simulink model "LunarMicrogrid_Full"  (R2026b)
settings: Solver=ode23t  StopTime=simulation.timeSim  MaxStep=1/(5*solarPlant.converterSwitchingFrequency)  AbsTol=1e-3
PreLoadFcn:
  | run('LunarMicrogridA_Data');
values from neighbouring files (symbols this model uses):
  Csc = Csc_cell/Ns_sc*Np_sc    (= 200)    [LunarDAB_Params.m]
  eta_sc = 0.95    [LunarDAB_Params.m]
  fsw = 100e3    (= 100000)    [LunarDAB_Params.m]
  k_restore = 1    [LunarDAB_Params.m]
  kiCurrent = 2    [LunarDAB_Params.m]
  kiVoltage = 8    [LunarDAB_Params.m]
  kpCurrent = 0.005    [LunarDAB_Params.m]
  kpVoltage = 0.4    [LunarDAB_Params.m]
  lTotal = lSeries + Llk    [LunarDAB_Params.m]
  P170_dt = 1e-4    (= 0.0001)    [P170_PV_Initialize.m]
  P170_Imp = im(ix)    [P170_PV_Initialize.m]
  P170_Vmp = vm(ix)    [P170_PV_Initialize.m]
  Rd_bat = dV_droop/Ibat_max    (= 0.232258064516)    [LunarDAB_Params.m]
  SC_enable = 1    [LunarDAB_Params.m]
  thetaIC = 0    [LunarDAB_Params.m]
  thetaMaxDab = pi/4    (= 0.785398163397)    [LunarDAB_Params.m]
  Tsw = 1/fsw    (= 1e-05)    [LunarDAB_Params.m]
  Vsc0 = sqrt((Vsc_max^2 + Vsc_min^2)/2)    [LunarDAB_Params.m]
  Vsc_max = 119    [LunarDAB_Params.m]
  Vsc_min = 66    [LunarDAB_Params.m]
undefined symbols (not defined in the file or in its folder): a_lpf_sys, battery, bms, connectedLoad, dcVoltage, DiscIntNeverNeededParam, eta_dab, Ibat_sign, mmc, Ndab, P170_T, pvDroop, sc, sensor, socLimit, solarPlant
libraries: sl_discontinuities x13, fl_lib x13, nesl_utility x13, simulink x7, batteryecm_lib x1, simulink_extras x1, ee_lib x1
(part 7 of 8)

== system LunarMicrogrid_Full/BESS Controller/PIctrl/Filter/Disc. Forward Euler Filter ==
  U : Inport  SampleTime=SampleTime
  Nout : Inport  Port=2  SampleTime=SampleTime
  Reset : Inport  Port=3  SampleTime=SampleTime
  D0in : Inport  Port=4  SampleTime=SampleTime
  N : Inport  Port=5  SampleTime=SampleTime
  Ts : Inport  Port=6  SampleTime=SampleTime
  Filter : DiscreteIntegrator  DisableCoverage=on  SampleTime=SampleTime  OutMin=FilterOutMin  OutMax=FilterOutMax  RndMeth=Simplest  ICPrevOutput=DiscIntNeverNeededParam  ICPrevScaledInput=DiscIntNeverNeededParam
  Signal Specification2 : SignalSpecification  DisableCoverage=on  OutDataTypeStr=boolean  SampleTime=SampleTime
  SumD : Sum  DisableCoverage=on  Inputs=|+-  OutMin=SumDOutMin  OutMax=SumDOutMax  RndMeth=Simplest
  Terminator{,1..3} (4 alike) : Terminator
  Y : Outport  SampleTime=SampleTime
  wires:
  Ts/1 -> Terminator3/1
  D0in/1 -> Terminator/1
  SumD/1 -> Y/1
  Nout/1 -> Filter/1
  U/1 -> SumD/1
  Filter/1 -> SumD/2
  N/1 -> Signal Specification2/1
  Signal Specification2/1 -> Terminator2/1
  Reset/1 -> Terminator1/1

== system LunarMicrogrid_Full/BESS Controller/PIctrl/Filter/Disc. Forward Euler Filter Only ==
  U : Inport  SampleTime=SampleTime
  Nout : Inport  Port=2  SampleTime=SampleTime
  Reset : Inport  Port=3  SampleTime=SampleTime
  D0in : Inport  Port=4  SampleTime=SampleTime
  N : Inport  Port=5  SampleTime=SampleTime
  Ts : Inport  Port=6  SampleTime=SampleTime
  Filter : DiscreteIntegrator  DisableCoverage=on  InitialCondition=InitialConditionForFilter  SampleTime=SampleTime  OutMin=FilterOutMin  OutMax=FilterOutMax  ICPrevOutput=DiscIntNeverNeededParam  ICPrevScaledInput=DiscIntNeverNeededParam
  Signal Specification2 : SignalSpecification  DisableCoverage=on  OutDataTypeStr=boolean  SampleTime=SampleTime
  SumD : Sum  DisableCoverage=on  Inputs=|+-  OutMin=SumDOutMin  OutMax=SumDOutMax
  Terminator{,1..3} (4 alike) : Terminator
  Y : Outport  SampleTime=SampleTime
  wires:
  Filter/1 -> Y/1
  Reset/1 -> Terminator1/1
  Signal Specification2/1 -> Terminator2/1
  N/1 -> Signal Specification2/1
  Nout/1 -> SumD/2
  U/1 -> SumD/1
  SumD/1 -> Filter/1
  D0in/1 -> Terminator/1
  Ts/1 -> Terminator3/1

== system LunarMicrogrid_Full/BESS Controller/PIctrl/Filter/Disc. Trapezoidal Filter ==
  note: Denominator Coefficients
  U : Inport  SampleTime=SampleTime
  N : Inport  Port=2  SampleTime=SampleTime
  Reset : Inport  Port=3  SampleTime=SampleTime
  D0in : Inport  Port=4  SampleTime=SampleTime
  Nout : Inport  Port=5  SampleTime=SampleTime
  Ts : Inport  Port=6  SampleTime=SampleTime
  DenCoefOut : Product  OutMin=FilterDiffOutCoefMin  OutMax=FilterDiffOutCoefMax  RndMeth=Simplest  SampleTime=SampleTime
  Divide : Product  InputSameDT=on  OutMin=DivideOutMin  OutMax=DivideOutMax  RndMeth=Simplest  SampleTime=SampleTime
  Filter Den Constant : Constant  DisableCoverage=on  OutMin=FilterDenConstantOutMin  OutMax=FilterDenConstantOutMax  OutDataTypeStr=Inherit: Inherit via back propagation  PreserveConstantTs=on
  Filter Differentiator TF : DiscreteTransferFcn  Numerator=[1 -1]  DenominatorSource=Input port  SampleTime=SampleTime  a0EqualsOne=on  RndMeth=Simplest
      settings: InputPortMap=u0,p3
  Mux : Mux  Inputs=2
  Passthrough for tuning : DataTypeConversion  Tag=#GainSurfaceTarget_  RndMeth=Simplest  SaturateOnIntegerOverflow=off
  Reciprocal : Math  Operator=reciprocal  OutMin=ReciprocalOutMin  OutMax=ReciprocalOutMax  RndMeth=Simplest  SaturateOnIntegerOverflow=off  OutDataTypeStr=Inherit: Inherit via internal rule
  SumDen : Sum  Inputs=++|  OutMin=SumDenOutMin  OutMax=SumDenOutMax  InputSameDT=on  RndMeth=Simplest
  SumNum : Sum  Inputs=-+|  OutMin=SumNumOutMin  OutMax=SumNumOutMax  InputSameDT=on  RndMeth=Simplest
  Terminator : Terminator
  Terminator1 : Terminator
  Terminator2 : Terminator
  Tsamp : Subsystem  Variant=on  VariantControlMode=label  LabelModeActiveChoice=InternalTs
  Y : Outport  SampleTime=SampleTime
  wires:
  Ts/1 -> Tsamp/2(Ts)
  D0in/1 -> Terminator/1
  Passthrough for tuning/1 -> Tsamp/1(N)
  Tsamp/1(Out1) -> SumDen/2, SumNum/2
  Filter Den Constant/1 -> SumNum/1, Mux/1, SumDen/1
  SumDen/1 -> Reciprocal/1
  SumNum/1 -> Divide/2
  Divide/1 -> Mux/2
  Reciprocal/1 -> DenCoefOut/2, Divide/1
  U/1 -> Filter Differentiator TF/1
  Filter Differentiator TF/1 -> DenCoefOut/1
  Mux/1 -> Filter Differentiator TF/2
  N/1 -> Passthrough for tuning/1
  DenCoefOut/1 -> Y/1
  Nout/1 -> Terminator2/1
  Reset/1 -> Terminator1/1

== system LunarMicrogrid_Full/BESS Controller/PIctrl/Filter/Disc. Trapezoidal Filter Only ==
  note: Denominator Coefficients
  U : Inport  SampleTime=SampleTime
  N : Inport  Port=2  SampleTime=SampleTime
  Reset : Inport  Port=3  SampleTime=SampleTime
  D0in : Inport  Port=4  SampleTime=SampleTime
  Nout : Inport  Port=5  SampleTime=SampleTime
  Ts : Inport  Port=6  SampleTime=SampleTime
  DenCoefOut : Product  OutMin=FilterDiffOutCoefMin  OutMax=FilterDiffOutCoefMax  SampleTime=SampleTime
  Filter Den Constant : Constant  DisableCoverage=on  Value=2  OutMin=FilterDenConstantOutMin  OutMax=FilterDenConstantOutMax  OutDataTypeStr=Inherit: Inherit via back propagation  PreserveConstantTs=on
  Filter Differentiator TF : DiscreteTransferFcn  Numerator=[1 1]  DenominatorSource=Input port  InitialStates=InitialConditionForFilter  SampleTime=SampleTime  a0EqualsOne=on
      settings: InputPortMap=u0,p3
  Mux : Mux  Inputs=2
  Passthrough for tuning : DataTypeConversion  Tag=#GainSurfaceTarget_  SaturateOnIntegerOverflow=off  RndMeth=Floor
  SumDen : Sum  Inputs=|++  OutMin=SumDenOutMin  OutMax=SumDenOutMax  InputSameDT=on
  SumNum : Sum  Inputs=-+|  OutMin=SumNumOutMin  OutMax=SumNumOutMax  InputSameDT=on
  Terminator : Terminator
  Terminator1 : Terminator
  Terminator2 : Terminator
  Tsamp : Subsystem  Variant=on  VariantControlMode=label  LabelModeActiveChoice=InternalTs
  Y : Outport  SampleTime=SampleTime
  wires:
  SumNum/1 -> Mux/2
  SumDen/1 -> Mux/1
  Filter Den Constant/1 -> SumDen/1, SumNum/1
  Tsamp/1(Out1) -> SumDen/2, SumNum/2, DenCoefOut/2
  Reset/1 -> Terminator1/1
  Nout/1 -> Terminator2/1
  DenCoefOut/1 -> Y/1
  N/1 -> Passthrough for tuning/1
  Mux/1 -> Filter Differentiator TF/2
  Filter Differentiator TF/1 -> DenCoefOut/1
  U/1 -> Filter Differentiator TF/1
  Passthrough for tuning/1 -> Tsamp/1(N)
  D0in/1 -> Terminator/1
  Ts/1 -> Tsamp/2(Ts)

== system LunarMicrogrid_Full/BESS Controller/PIctrl/Filter/Passthrough ==
  Reset : Inport  SampleTime=SampleTime
  U : Inport  Port=2  SampleTime=SampleTime
  N : Inport  Port=3  SampleTime=SampleTime
  D0in : Inport  Port=4  SampleTime=SampleTime
  Nout : Inport  Port=5  SampleTime=SampleTime
  Ts : Inport  Port=6  SampleTime=SampleTime
  Signal Specification1 : SignalSpecification  DisableCoverage=on  OutDataTypeStr=boolean  SampleTime=SampleTime
  Signal Specification4 : SignalSpecification  DisableCoverage=on  OutDataTypeStr=boolean  SampleTime=SampleTime
  Terminator{1..2,4..6} (5 alike) : Terminator
  Y : Outport  SampleTime=SampleTime
  wires:
  Nout/1 -> Terminator2/1
  Reset/1 -> Terminator5/1
  D0in/1 -> Signal Specification4/1
  Signal Specification4/1 -> Terminator4/1
  N/1 -> Signal Specification1/1
  Signal Specification1/1 -> Terminator1/1
  U/1 -> Y/1
  Ts/1 -> Terminator6/1

== system LunarMicrogrid_Full/BESS Controller/PIctrl/Filter ICs/Disabled ==
  D0 : Inport  SampleTime=SampleTime
  Ground : Ground  DisableCoverage=on
  Signal Specification : SignalSpecification  DisableCoverage=on  OutDataTypeStr=boolean  SampleTime=SampleTime
  Signal Specification1 : SignalSpecification  DisableCoverage=on  OutDataTypeStr=boolean  SampleTime=SampleTime
  Terminator : Terminator
  Out1 : Outport  SampleTime=SampleTime
  wires:
  D0/1 -> Signal Specification/1
  Signal Specification/1 -> Terminator/1
  Ground/1 -> Signal Specification1/1
  Signal Specification1/1 -> Out1/1

== system LunarMicrogrid_Full/BESS Controller/PIctrl/Filter ICs/External IC ==
  D0 : Inport  SampleTime=SampleTime
  Out1 : Outport  SampleTime=SampleTime
  wires:
  D0/1 -> Out1/1

== system LunarMicrogrid_Full/BESS Controller/PIctrl/Filter ICs/Internal IC - Differentiator ==
  D0 : Inport  SampleTime=SampleTime
  Ground : Ground  DisableCoverage=on
  Signal Specification : SignalSpecification  DisableCoverage=on  OutDataTypeStr=boolean  SampleTime=SampleTime
  Signal Specification1 : SignalSpecification  DisableCoverage=on  OutDataTypeStr=boolean  SampleTime=SampleTime
  Terminator : Terminator
  Out1 : Outport  SampleTime=SampleTime
  wires:
  D0/1 -> Signal Specification/1
  Signal Specification/1 -> Terminator/1
  Ground/1 -> Signal Specification1/1
  Signal Specification1/1 -> Out1/1

== system LunarMicrogrid_Full/BESS Controller/PIctrl/Filter ICs/Internal IC - Filter ==
  D0 : Inport  SampleTime=SampleTime
  Ground : Ground  DisableCoverage=on
  Signal Specification : SignalSpecification  DisableCoverage=on  OutDataTypeStr=boolean  SampleTime=SampleTime
  Signal Specification1 : SignalSpecification  DisableCoverage=on  OutDataTypeStr=boolean  SampleTime=SampleTime
  Terminator : Terminator
  Out1 : Outport  SampleTime=SampleTime
  wires:
  D0/1 -> Signal Specification/1
  Signal Specification/1 -> Terminator/1
  Ground/1 -> Signal Specification1/1
  Signal Specification1/1 -> Out1/1

== system LunarMicrogrid_Full/BESS Controller/PIctrl/I Gain/Disabled ==
  I Gain : Inport  SampleTime=SampleTime
  Signal Specification : SignalSpecification  DisableCoverage=on  OutDataTypeStr=boolean  SampleTime=SampleTime
  Terminator : Terminator
  wires:
  Signal Specification/1 -> Terminator/1
  I Gain/1 -> Signal Specification/1

== system LunarMicrogrid_Full/BESS Controller/PIctrl/I Gain/External Parameters ==
  err : Inport  SampleTime=SampleTime
  I Gain : Inport  Port=2  SampleTime=SampleTime
  IProd Out : Product  OutMin=IOutMin  OutMax=IOutMax  RndMeth=Simplest  SampleTime=SampleTime  OutDataTypeStr=Inherit: Same as first input
  Out1 : Outport  SampleTime=SampleTime
  wires:
  err/1 -> IProd Out/1
  I Gain/1 -> IProd Out/2
  IProd Out/1 -> Out1/1

== system LunarMicrogrid_Full/BESS Controller/PIctrl/I Gain/Internal Parameters ==
  err : Inport  SampleTime=SampleTime
  I Gain : Inport  Port=2  SampleTime=SampleTime
  Integral Gain : Gain  DisableCoverage=on  Gain=I  ParamMin=IParamMin  ParamMax=IParamMax  OutMin=IOutMin  OutMax=IOutMax  RndMeth=Simplest  OutDataTypeStr=Inherit: Same as input
  Signal Specification : SignalSpecification  DisableCoverage=on  OutDataTypeStr=boolean  SampleTime=SampleTime
  Terminator : Terminator
  Out1 : Outport  SampleTime=SampleTime
  wires:
  err/1 -> Integral Gain/1
  Integral Gain/1 -> Out1/1
  Signal Specification/1 -> Terminator/1
  I Gain/1 -> Signal Specification/1

== system LunarMicrogrid_Full/BESS Controller/PIctrl/Ideal P Gain/External Parameters ==
  In1 : Inport  SampleTime=SampleTime
  P Gain : Inport  Port=2  SampleTime=SampleTime
  PProd Out : Product  RndMeth=Simplest  SampleTime=SampleTime  OutDataTypeStr=Inherit: Same as first input
  Out1 : Outport  SampleTime=SampleTime
  wires:
  In1/1 -> PProd Out/1
  P Gain/1 -> PProd Out/2
  PProd Out/1 -> Out1/1

== system LunarMicrogrid_Full/BESS Controller/PIctrl/Ideal P Gain/Internal Parameters ==
  In1 : Inport  SampleTime=SampleTime
  P Gain : Inport  Port=2  SampleTime=SampleTime
  Proportional Gain : Gain  Gain=P  ParamMin=PParamMin  ParamMax=PParamMax  OutMin=POutMin  OutMax=POutMax  RndMeth=Simplest  OutDataTypeStr=Inherit: Same as input
  Signal Specification1 : SignalSpecification  DisableCoverage=on  OutDataTypeStr=boolean  SampleTime=SampleTime
  Terminator1 : Terminator
  Out1 : Outport  SampleTime=SampleTime
  wires:
  In1/1 -> Proportional Gain/1
  Proportional Gain/1 -> Out1/1
  P Gain/1 -> Signal Specification1/1
  Signal Specification1/1 -> Terminator1/1

== system LunarMicrogrid_Full/BESS Controller/PIctrl/Ideal P Gain/Passthrough ==
  In1 : Inport  SampleTime=SampleTime
  P Gain : Inport  Port=2  SampleTime=SampleTime
  Terminator1 : Terminator
  Out1 : Outport  SampleTime=SampleTime
  wires:
  In1/1 -> Out1/1
  P Gain/1 -> Terminator1/1

== system LunarMicrogrid_Full/BESS Controller/PIctrl/Ideal P Gain Fdbk/Disabled ==
  In1 : Inport  SampleTime=SampleTime
  P Gain : Inport  Port=2  SampleTime=SampleTime
  Signal Specification1 : SignalSpecification  DisableCoverage=on  OutDataTypeStr=boolean  SampleTime=SampleTime
  Terminator1 : Terminator
  Terminator2 : Terminator
  wires:
  P Gain/1 -> Terminator1/1
  In1/1 -> Signal Specification1/1
  Signal Specification1/1 -> Terminator2/1

== system LunarMicrogrid_Full/BESS Controller/PIctrl/Ideal P Gain Fdbk/External Parameters ==
  In1 : Inport  SampleTime=SampleTime
  P Gain : Inport  Port=2  SampleTime=SampleTime
  PProd Out : Product  RndMeth=Simplest  SampleTime=SampleTime  OutDataTypeStr=Inherit: Same as first input
  Out1 : Outport  SampleTime=SampleTime
  wires:
  PProd Out/1 -> Out1/1
  P Gain/1 -> PProd Out/2
  In1/1 -> PProd Out/1

== system LunarMicrogrid_Full/BESS Controller/PIctrl/Ideal P Gain Fdbk/Internal Parameters ==
  In1 : Inport  SampleTime=SampleTime
  P Gain : Inport  Port=2  SampleTime=SampleTime
  Proportional Gain : Gain  Gain=P  ParamMin=PParamMin  ParamMax=PParamMax  OutMin=POutMin  OutMax=POutMax  RndMeth=Simplest  OutDataTypeStr=Inherit: Same as input
  Signal Specification1 : SignalSpecification  DisableCoverage=on  OutDataTypeStr=boolean  SampleTime=SampleTime
  Terminator1 : Terminator
  Out1 : Outport  SampleTime=SampleTime
  wires:
  Proportional Gain/1 -> Out1/1
  In1/1 -> Proportional Gain/1
  Signal Specification1/1 -> Terminator1/1
  P Gain/1 -> Signal Specification1/1

== system LunarMicrogrid_Full/BESS Controller/PIctrl/Ideal P Gain Fdbk/Passthrough ==
  In1 : Inport  SampleTime=SampleTime
  P Gain : Inport  Port=2  SampleTime=SampleTime
  Terminator1 : Terminator
  Out1 : Outport  SampleTime=SampleTime
  wires:
  In1/1 -> Out1/1
  P Gain/1 -> Terminator1/1

== system LunarMicrogrid_Full/BESS Controller/PIctrl/Integrator/Continuous ==
  U : Inport  SampleTime=SampleTime
  Reset : Inport  Port=2  SampleTime=SampleTime
  I0in : Inport  Port=3  SampleTime=SampleTime
  Ground : Ground  DisableCoverage=on
  Integrator : Integrator
  Signal Specification1 : SignalSpecification  DisableCoverage=on  OutDataTypeStr=boolean  SampleTime=SampleTime
  Terminator : Terminator
  Terminator1 : Terminator
  state : Outport  SampleTime=SampleTime
  out : Outport  Port=2  SampleTime=SampleTime
  wires:
  U/1 -> Integrator/1
  I0in/1 -> Terminator/1
  Integrator/1 -> out/1
  Ground/1 -> Signal Specification1/1
  Signal Specification1/1 -> state/1
  Reset/1 -> Terminator1/1

== system LunarMicrogrid_Full/BESS Controller/PIctrl/Integrator/Disabled ==
  U : Inport  SampleTime=SampleTime
  Reset : Inport  Port=2  SampleTime=SampleTime
  I0in : Inport  Port=3  SampleTime=SampleTime
  Ground : Ground  DisableCoverage=on
  Signal Specification1 : SignalSpecification  DisableCoverage=on  OutDataTypeStr=boolean  SampleTime=SampleTime
  Signal Specification2 : SignalSpecification  DisableCoverage=on  OutDataTypeStr=boolean  SampleTime=SampleTime
  Signal Specification4 : SignalSpecification  DisableCoverage=on  OutDataTypeStr=boolean  SampleTime=SampleTime
  Terminator1 : Terminator
  Terminator2 : Terminator
  Terminator3 : Terminator
  out : Outport  SampleTime=SampleTime
  wires:
  Reset/1 -> Terminator2/1
  Signal Specification4/1 -> Terminator1/1
  I0in/1 -> Signal Specification4/1
  U/1 -> Signal Specification1/1
  Signal Specification1/1 -> Terminator3/1
  Ground/1 -> Signal Specification2/1
  Signal Specification2/1 -> out/1

== system LunarMicrogrid_Full/BESS Controller/PIctrl/Integrator/Discrete ==
  U : Inport  SampleTime=SampleTime
  Reset : Inport  Port=2  SampleTime=SampleTime
  I0in : Inport  Port=3  SampleTime=SampleTime
  Ground_Integrator : Ground  DisableCoverage=on
  Integrator : DiscreteIntegrator  InitialCondition=thetaIC  SampleTime=SampleTime  OutMin=IntegratorOutMin  OutMax=IntegratorOutMax  RndMeth=Simplest  ICPrevOutput=DiscIntNeverNeededParam  ICPrevScaledInput=DiscIntNeverNeededParam
  Signal Specification1 : SignalSpecification  DisableCoverage=on  OutDataTypeStr=boolean  SampleTime=SampleTime
  Terminator : Terminator
  Terminator1 : Terminator
  Terminator2 : Terminator
  out : Outport  SampleTime=SampleTime
  state : Outport  Port=2  SampleTime=SampleTime
  wires:
  I0in/1 -> Terminator1/1
  Integrator/1 -> out/1
  U/1 -> Integrator/1
  Ground_Integrator/1 -> state/1, Signal Specification1/1
  Signal Specification1/1 -> Terminator/1
  Reset/1 -> Terminator2/1

== system LunarMicrogrid_Full/BESS Controller/PIctrl/Integrator ICs/Disabled ==
  I0 : Inport  SampleTime=SampleTime
  Ground : Ground  DisableCoverage=on
  Signal Specification : SignalSpecification  DisableCoverage=on  OutDataTypeStr=boolean  SampleTime=SampleTime
  Signal Specification1 : SignalSpecification  DisableCoverage=on  OutDataTypeStr=boolean  SampleTime=SampleTime
  Terminator : Terminator
  Out1 : Outport  SampleTime=SampleTime
  wires:
  Signal Specification/1 -> Terminator/1
  I0/1 -> Signal Specification/1
  Signal Specification1/1 -> Out1/1
  Ground/1 -> Signal Specification1/1

== system LunarMicrogrid_Full/BESS Controller/PIctrl/Integrator ICs/External IC ==
  I0 : Inport  SampleTime=SampleTime
  Out1 : Outport  SampleTime=SampleTime
  wires:
  I0/1 -> Out1/1

== system LunarMicrogrid_Full/BESS Controller/PIctrl/Integrator ICs/Internal IC ==
  I0 : Inport  SampleTime=SampleTime
  Ground : Ground  DisableCoverage=on
  Signal Specification : SignalSpecification  DisableCoverage=on  OutDataTypeStr=boolean  SampleTime=SampleTime
  Signal Specification1 : SignalSpecification  DisableCoverage=on  OutDataTypeStr=boolean  SampleTime=SampleTime
  Terminator : Terminator
  Out1 : Outport  SampleTime=SampleTime
  wires:
  I0/1 -> Signal Specification/1
  Signal Specification/1 -> Terminator/1
  Ground/1 -> Signal Specification1/1
  Signal Specification1/1 -> Out1/1

== system LunarMicrogrid_Full/BESS Controller/PIctrl/N Copy/Disabled ==
  N Gain : Inport  SampleTime=SampleTime
  Terminator : Terminator
  wires:
  N Gain/1 -> Terminator/1

== system LunarMicrogrid_Full/BESS Controller/PIctrl/N Copy/Disabled wSignal Specification ==
  N Gain : Inport  SampleTime=SampleTime
  Signal Specification1 : SignalSpecification  DisableCoverage=on  OutDataTypeStr=boolean  SampleTime=SampleTime
  Terminator : Terminator
  wires:
  N Gain/1 -> Signal Specification1/1
  Signal Specification1/1 -> Terminator/1

== system LunarMicrogrid_Full/BESS Controller/PIctrl/N Copy/External Parameters ==
  N Gain : Inport  SampleTime=SampleTime
  Out1 : Outport  SampleTime=SampleTime
  wires:
  N Gain/1 -> Out1/1

== system LunarMicrogrid_Full/BESS Controller/PIctrl/N Copy/Internal Parameters ==
  N Gain : Inport  SampleTime=SampleTime
  N Copy : Constant  DisableCoverage=on  Value=N  OutMin=NCopyOutMin  OutMax=NCopyOutMax  OutDataTypeStr=Inherit: Inherit via back propagation  PreserveConstantTs=on
  Signal Specification : SignalSpecification  DisableCoverage=on  OutDataTypeStr=boolean  SampleTime=SampleTime
  Terminator : Terminator
  Out1 : Outport  SampleTime=SampleTime
  wires:
  N Copy/1 -> Out1/1
  N Gain/1 -> Signal Specification/1
  Signal Specification/1 -> Terminator/1

== system LunarMicrogrid_Full/BESS Controller/PIctrl/N Gain/Disabled ==
  U : Inport  SampleTime=SampleTime
  N Gain : Inport  Port=2  SampleTime=SampleTime
  Signal Specification1 : SignalSpecification  DisableCoverage=on  OutDataTypeStr=boolean  SampleTime=SampleTime
  Signal Specification2 : SignalSpecification  DisableCoverage=on  OutDataTypeStr=boolean  SampleTime=SampleTime
  Terminator1 : Terminator
  Terminator2 : Terminator
  wires:
  Signal Specification2/1 -> Terminator2/1
  U/1 -> Signal Specification2/1
  N Gain/1 -> Signal Specification1/1
  Signal Specification1/1 -> Terminator1/1

== system LunarMicrogrid_Full/BESS Controller/PIctrl/N Gain/External Parameters ==
  U : Inport  SampleTime=SampleTime
  N Gain : Inport  Port=2  SampleTime=SampleTime
  NProd Out : Product  OutMin=NOutMin  OutMax=NOutMax  RndMeth=Simplest  SampleTime=SampleTime
  Out1 : Outport  SampleTime=SampleTime
  wires:
  U/1 -> NProd Out/1
  N Gain/1 -> NProd Out/2
  NProd Out/1 -> Out1/1

== system LunarMicrogrid_Full/BESS Controller/PIctrl/N Gain/Internal Parameters ==
  U : Inport  SampleTime=SampleTime
  N Gain : Inport  Port=2  SampleTime=SampleTime
  Filter Coefficient : Gain  Gain=N  ParamMin=NParamMin  ParamMax=NParamMax  OutMin=NOutMin  OutMax=NOutMax  RndMeth=Simplest
  Signal Specification1 : SignalSpecification  DisableCoverage=on  OutDataTypeStr=boolean  SampleTime=SampleTime
  Terminator1 : Terminator
  Out1 : Outport  SampleTime=SampleTime
  wires:
  U/1 -> Filter Coefficient/1
  Filter Coefficient/1 -> Out1/1
  N Gain/1 -> Signal Specification1/1
  Signal Specification1/1 -> Terminator1/1

== system LunarMicrogrid_Full/BESS Controller/PIctrl/N Gain/Passthrough ==
  U : Inport  SampleTime=SampleTime
  N Gain : Inport  Port=2  SampleTime=SampleTime
  Terminator1 : Terminator
  Out1 : Outport  SampleTime=SampleTime
  wires:
  U/1 -> Out1/1
  N Gain/1 -> Terminator1/1

== system LunarMicrogrid_Full/BESS Controller/PIctrl/P Copy/Disabled ==
  P Gain : Inport  SampleTime=SampleTime
  Terminator3 : Terminator
  wires:
  P Gain/1 -> Terminator3/1

== system LunarMicrogrid_Full/BESS Controller/PIctrl/P Copy/External Parameters Ideal ==
  P Gain : Inport  SampleTime=SampleTime
  Out1 : Outport  SampleTime=SampleTime
  wires:
  P Gain/1 -> Out1/1

== system LunarMicrogrid_Full/BESS Controller/PIctrl/P Copy/Internal Parameters Ideal ==
  P Gain : Inport  SampleTime=SampleTime
  P Copy : Constant  DisableCoverage=on  Value=P  OutMin=PCopyOutMin  OutMax=PCopyOutMax  OutDataTypeStr=Inherit: Inherit via back propagation  PreserveConstantTs=on
  Terminator3 : Terminator
  Out1 : Outport  SampleTime=SampleTime
  wires:
  P Copy/1 -> Out1/1
  P Gain/1 -> Terminator3/1

== system LunarMicrogrid_Full/BESS Controller/PIctrl/Parallel P Gain/Disabled ==
  P Gain : Inport  SampleTime=SampleTime
  Signal Specification : SignalSpecification  DisableCoverage=on  OutDataTypeStr=boolean  SampleTime=SampleTime
  Terminator : Terminator
  wires:
  P Gain/1 -> Signal Specification/1
  Signal Specification/1 -> Terminator/1

== system LunarMicrogrid_Full/BESS Controller/PIctrl/Parallel P Gain/External Parameters ==
  err : Inport  SampleTime=SampleTime
  P Gain : Inport  Port=2  SampleTime=SampleTime
  PProd Out : Product  OutMin=POutMin  OutMax=POutMax  RndMeth=Simplest  SampleTime=SampleTime  OutDataTypeStr=Inherit: Same as first input
  Out1 : Outport  SampleTime=SampleTime
  wires:
  PProd Out/1 -> Out1/1
  P Gain/1 -> PProd Out/2
  err/1 -> PProd Out/1

== system LunarMicrogrid_Full/BESS Controller/PIctrl/Parallel P Gain/Internal Parameters ==
  err : Inport  SampleTime=SampleTime
  P Gain : Inport  Port=2  SampleTime=SampleTime
  Proportional Gain : Gain  Gain=P  ParamMin=PParamMin  ParamMax=PParamMax  OutMin=POutMin  OutMax=POutMax  RndMeth=Simplest  OutDataTypeStr=Inherit: Same as input
  Signal Specification : SignalSpecification  DisableCoverage=on  OutDataTypeStr=boolean  SampleTime=SampleTime
  Terminator : Terminator
  Out1 : Outport  SampleTime=SampleTime
  wires:
  Proportional Gain/1 -> Out1/1
  err/1 -> Proportional Gain/1
  Signal Specification/1 -> Terminator/1
  P Gain/1 -> Signal Specification/1

== system LunarMicrogrid_Full/BESS Controller/PIctrl/Parallel P Gain/Passthrough ==
  err : Inport  SampleTime=SampleTime
  P Gain : Inport  Port=2  SampleTime=SampleTime
  Terminator : Terminator
  Out1 : Outport  SampleTime=SampleTime
  wires:
  err/1 -> Out1/1
  P Gain/1 -> Terminator/1

== system LunarMicrogrid_Full/BESS Controller/PIctrl/Reset Signal/Disabled ==
  Reset : Inport  SampleTime=SampleTime
  Ground : Ground  DisableCoverage=on
  Signal Specification : SignalSpecification  DisableCoverage=on  OutDataTypeStr=boolean  SampleTime=SampleTime
  Signal Specification1 : SignalSpecification  DisableCoverage=on  OutDataTypeStr=boolean  SampleTime=SampleTime
  Terminator : Terminator
  Out1 : Outport  SampleTime=SampleTime
  wires:
  Reset/1 -> Signal Specification/1
  Signal Specification/1 -> Terminator/1
  Ground/1 -> Signal Specification1/1
  Signal Specification1/1 -> Out1/1

== system LunarMicrogrid_Full/BESS Controller/PIctrl/Reset Signal/External Reset ==
  Reset : Inport  SampleTime=SampleTime
  Out1 : Outport  SampleTime=SampleTime
  wires:
  Reset/1 -> Out1/1

== system LunarMicrogrid_Full/BESS Controller/PIctrl/Saturation/Enabled ==
  In1 : Inport  SampleTime=SampleTime
  Upper Limit : Inport  Port=2  SampleTime=SampleTime
  Lower Limit : Inport  Port=3  SampleTime=SampleTime
  Saturation : Saturate  UpperLimit=UpperSaturationLimit  LowerLimit=LowerSaturationLimit  LinearizeAsGain=off  SampleTime=SampleTime  OutMin=SaturationOutMin  OutMax=SaturationOutMax  OutDataTypeStr=Inherit: Inherit via back propagation  RndMeth=Simplest
  Signal Specification : SignalSpecification  DisableCoverage=on  OutDataTypeStr=boolean  SampleTime=SampleTime
  Signal Specification1 : SignalSpecification  DisableCoverage=on  OutDataTypeStr=boolean  SampleTime=SampleTime
  Terminator : Terminator
  Terminator1 : Terminator
  Out1 : Outport  SampleTime=SampleTime
  wires:
  Signal Specification1/1 -> Terminator1/1
  Upper Limit/1 -> Signal Specification/1
  Lower Limit/1 -> Signal Specification1/1
  Signal Specification/1 -> Terminator/1
  In1/1 -> Saturation/1
  Saturation/1 -> Out1/1

== system LunarMicrogrid_Full/BESS Controller/PIctrl/Saturation/External ==
  In1 : Inport  SampleTime=SampleTime
  Upper Limit : Inport  Port=2  SampleTime=SampleTime
  Lower Limit : Inport  Port=3  SampleTime=SampleTime
  Saturation Dynamic : sl_discontinuities/Saturation Dynamic  OutMin=SaturationOutMin  OutMax=SaturationOutMax  OutDataTypeStr=Inherit: Same as second input  OutDataType=fixdt(1, 16)  OutScaling=2^-10  RndMeth=Simplest  DoSatur=off
  Out1 : Outport  SampleTime=SampleTime
  wires:
  Lower Limit/1 -> Saturation Dynamic/3
  Upper Limit/1 -> Saturation Dynamic/1
  Saturation Dynamic/1 -> Out1/1
  In1/1 -> Saturation Dynamic/2

== system LunarMicrogrid_Full/BESS Controller/PIctrl/Saturation/Passthrough ==
  In1 : Inport  SampleTime=SampleTime
  Upper Limit : Inport  Port=2  SampleTime=SampleTime
  Lower Limit : Inport  Port=3  SampleTime=SampleTime
  Signal Specification : SignalSpecification  DisableCoverage=on  OutDataTypeStr=boolean  SampleTime=SampleTime
  Signal Specification1 : SignalSpecification  DisableCoverage=on  OutDataTypeStr=boolean  SampleTime=SampleTime
  Terminator : Terminator
  Terminator1 : Terminator
  Out1 : Outport  SampleTime=SampleTime
  wires:
  Signal Specification1/1 -> Terminator1/1
  Lower Limit/1 -> Signal Specification1/1
  Upper Limit/1 -> Signal Specification/1
  Signal Specification/1 -> Terminator/1
  In1/1 -> Out1/1

== system LunarMicrogrid_Full/BESS Controller/PIctrl/Saturation Fdbk/Disabled ==
  In1 : Inport  SampleTime=SampleTime
  Signal Specification1 : SignalSpecification  DisableCoverage=on  OutDataTypeStr=boolean  SampleTime=SampleTime
  Terminator1 : Terminator
  wires:
  In1/1 -> Signal Specification1/1
  Signal Specification1/1 -> Terminator1/1

== system LunarMicrogrid_Full/BESS Controller/PIctrl/Saturation Fdbk/Enabled ==
  In1 : Inport  SampleTime=SampleTime
  Saturation : Saturate  UpperLimit=UpperSaturationLimit  LowerLimit=LowerSaturationLimit  LinearizeAsGain=off  SampleTime=SampleTime  OutMin=SaturationOutMin  OutMax=SaturationOutMax  OutDataTypeStr=Inherit: Inherit via back propagation  RndMeth=Simplest
  Out1 : Outport  SampleTime=SampleTime
  wires:
  Saturation/1 -> Out1/1
  In1/1 -> Saturation/1

== system LunarMicrogrid_Full/BESS Controller/PIctrl/Saturation Fdbk/External ==
  In1 : Inport  SampleTime=SampleTime
  Upper Limit : Inport  Port=2  SampleTime=SampleTime
  Lower Limit : Inport  Port=3  SampleTime=SampleTime
  Saturation Dynamic : sl_discontinuities/Saturation Dynamic  OutMin=SaturationOutMin  OutMax=SaturationOutMax  OutDataTypeStr=Inherit: Same as second input  OutDataType=fixdt(1, 16)  OutScaling=2^-10  RndMeth=Simplest  DoSatur=off
  Out1 : Outport  SampleTime=SampleTime
  wires:
  Lower Limit/1 -> Saturation Dynamic/3
  Upper Limit/1 -> Saturation Dynamic/1
  Saturation Dynamic/1 -> Out1/1
  In1/1 -> Saturation Dynamic/2

== system LunarMicrogrid_Full/BESS Controller/PIctrl/Saturation Fdbk/Passthrough ==
  In1 : Inport  SampleTime=SampleTime
  Out1 : Outport  SampleTime=SampleTime
  wires:
  In1/1 -> Out1/1

== system LunarMicrogrid_Full/BESS Controller/PIctrl/Sum/Passthrough_I ==
  P : Inport  SampleTime=SampleTime
  I : Inport  Port=2  SampleTime=SampleTime
  Signal Specification : SignalSpecification  OutDataTypeStr=boolean  SampleTime=SampleTime
  Terminator : Terminator
  Out1 : Outport  SampleTime=SampleTime
  wires:
  Signal Specification/1 -> Terminator/1
  P/1 -> Signal Specification/1
  I/1 -> Out1/1

== system LunarMicrogrid_Full/BESS Controller/PIctrl/Sum/Passthrough_P ==
  P : Inport  SampleTime=SampleTime
  Out1 : Outport  SampleTime=SampleTime
  wires:
  P/1 -> Out1/1

== system LunarMicrogrid_Full/BESS Controller/PIctrl/Sum/Sum_PD ==
  P : Inport  SampleTime=SampleTime
  D : Inport  Port=2  SampleTime=SampleTime
  Sum : Sum  Inputs=|++  OutMin=SumOutMin  OutMax=SumOutMax  RndMeth=Simplest  OutDataTypeStr=Inherit: Same as first input
  Out1 : Outport  SampleTime=SampleTime
  wires:
  P/1 -> Sum/1
  D/1 -> Sum/2
  Sum/1 -> Out1/1

== system LunarMicrogrid_Full/BESS Controller/PIctrl/Sum/Sum_PI ==
  P : Inport  SampleTime=SampleTime
  I : Inport  Port=2  SampleTime=SampleTime
  Sum : Sum  Inputs=|++  OutMin=SumOutMin  OutMax=SumOutMax  RndMeth=Simplest  OutDataTypeStr=Inherit: Same as first input
  Out1 : Outport  SampleTime=SampleTime
  wires:
  I/1 -> Sum/2
  P/1 -> Sum/1
  Sum/1 -> Out1/1

== system LunarMicrogrid_Full/BESS Controller/PIctrl/Sum/Sum_PID ==
  P : Inport  SampleTime=SampleTime
  I : Inport  Port=2  SampleTime=SampleTime
  D : Inport  Port=3  SampleTime=SampleTime
  Sum : Sum  Inputs=+++  OutMin=SumOutMin  OutMax=SumOutMax  RndMeth=Simplest  OutDataTypeStr=Inherit: Same as first input
  Out1 : Outport  SampleTime=SampleTime
  wires:
  I/1 -> Sum/2
  P/1 -> Sum/1
  D/1 -> Sum/3
  Sum/1 -> Out1/1

== system LunarMicrogrid_Full/BESS Controller/PIctrl/Sum Fdbk/Disabled ==
  fromP : Inport  SampleTime=SampleTime
  fromState : Inport  Port=2  SampleTime=SampleTime
  fromD : Inport  Port=3  SampleTime=SampleTime
  Signal Specification1 : SignalSpecification  DisableCoverage=on  OutDataTypeStr=boolean  SampleTime=SampleTime
  Terminator1 : Terminator
  Terminator2 : Terminator
  Terminator3 : Terminator
  wires:
  fromD/1 -> Terminator3/1
  fromState/1 -> Signal Specification1/1
  fromP/1 -> Terminator1/1
  Signal Specification1/1 -> Terminator2/1

== system LunarMicrogrid_Full/BESS Controller/PIctrl/Sum Fdbk/Enabled ==
  fromP : Inport  SampleTime=SampleTime
  fromState : Inport  Port=2  SampleTime=SampleTime
  fromD : Inport  Port=3  SampleTime=SampleTime
  Sum Fdbk : Sum  DisableCoverage=on  Inputs=+++  OutMin=SumOutMin  OutMax=SumOutMax  RndMeth=Simplest  OutDataTypeStr=Inherit: Same as first input
  Out1 : Outport  SampleTime=SampleTime
  wires:
  fromP/1 -> Sum Fdbk/1
  fromState/1 -> Sum Fdbk/2
  fromD/1 -> Sum Fdbk/3
  Sum Fdbk/1 -> Out1/1

== system LunarMicrogrid_Full/BESS Controller/PIctrl/Sum Fdbk/Passthrough ==
  fromState : Inport  SampleTime=SampleTime
  Out1 : Outport  SampleTime=SampleTime
  wires:
  fromState/1 -> Out1/1

== system LunarMicrogrid_Full/BESS Controller/PIctrl/Tracking Mode/Disabled ==
  uout : Inport  SampleTime=SampleTime
  TR : Inport  Port=2  SampleTime=SampleTime
  Signal Specification1 : SignalSpecification  DisableCoverage=on  OutDataTypeStr=boolean  SampleTime=SampleTime
  Terminator1 : Terminator
  Terminator3 : Terminator
  wires:
  uout/1 -> Terminator3/1
  TR/1 -> Signal Specification1/1
  Signal Specification1/1 -> Terminator1/1

== system LunarMicrogrid_Full/BESS Controller/PIctrl/Tracking Mode/Enabled ==
  uout : Inport  SampleTime=SampleTime
  TR : Inport  Port=2  SampleTime=SampleTime
  Kt : Gain  Gain=Kt  ParamMin=KtParamMin  ParamMax=KtParamMax  OutMin=KtOutMin  OutMax=KtOutMax  RndMeth=Simplest
  SumI3 : Sum  Inputs=|-+  OutMin=SumI3OutMin  OutMax=SumI3OutMax  RndMeth=Simplest
  Out1 : Outport  SampleTime=SampleTime
  wires:
  Kt/1 -> Out1/1
  SumI3/1 -> Kt/1
  TR/1 -> SumI3/2
  uout/1 -> SumI3/1

== system LunarMicrogrid_Full/BESS Controller/PIctrl/Tracking Mode Sum/Passthrough ==
  fromIgain : Inport  SampleTime=SampleTime
  fromTR : Inport  Port=2  SampleTime=SampleTime
  Signal Specification : SignalSpecification  DisableCoverage=on  OutDataTypeStr=boolean  SampleTime=SampleTime
  Terminator : Terminator
  preInt : Outport
  wires:
  fromIgain/1 -> preInt/1
  fromTR/1 -> Signal Specification/1
  Signal Specification/1 -> Terminator/1

== system LunarMicrogrid_Full/BESS Controller/PIctrl/Tracking Mode Sum/Tracking Mode ==
  fromIgain : Inport  SampleTime=SampleTime
  fromTR : Inport  Port=2  SampleTime=SampleTime
  SumI1 : Sum  Inputs=|++  OutMin=SumI1OutMin  OutMax=SumI1OutMax  RndMeth=Simplest
  preInt : Outport
  wires:
  fromIgain/1 -> SumI1/1
  fromTR/1 -> SumI1/2
  SumI1/1 -> preInt/1

== system LunarMicrogrid_Full/BESS Controller/PIctrl/Tsamp - Integral/Disabled ==
  U : Inport  SampleTime=SampleTime
  Ts : Inport  Port=2  SampleTime=SampleTime
  Terminator : Terminator
  Out1 : Outport  SampleTime=SampleTime
  wires:
  U/1 -> Out1/1
  Ts/1 -> Terminator/1

== system LunarMicrogrid_Full/BESS Controller/PIctrl/Tsamp - Integral/External Ts ==
  U : Inport  SampleTime=SampleTime
  Ts : Inport  Port=2  SampleTime=SampleTime
  Uintegral*Ts Prod Out : Product  OutMin=UintegralTsProdOutMin  OutMax=UintegralTsProdOutMax  RndMeth=Simplest  SampleTime=SampleTime
  Out1 : Outport  SampleTime=SampleTime
  wires:
  U/1 -> Uintegral*Ts Prod Out/1
  Uintegral*Ts Prod Out/1 -> Out1/1
  Ts/1 -> Uintegral*Ts Prod Out/2

== system LunarMicrogrid_Full/BESS Controller/PIctrl/Tsamp - Integral/Passthrough ==
  U : Inport  SampleTime=SampleTime
  Ts : Inport  Port=2  SampleTime=SampleTime
  Terminator : Terminator
  Out1 : Outport  SampleTime=SampleTime
  wires:
  Ts/1 -> Terminator/1
  U/1 -> Out1/1

== system LunarMicrogrid_Full/BESS Controller/PIctrl/Tsamp - Integral/TsSignalSpecification ==
  U : Inport  SampleTime=SampleTime
  Ts : Inport  Port=2  SampleTime=SampleTime
  Signal Specification : SignalSpecification  DisableCoverage=on  OutDataTypeStr=boolean  SampleTime=SampleTime
  Terminator : Terminator
  Out1 : Outport  SampleTime=SampleTime
  wires:
  U/1 -> Out1/1
  Ts/1 -> Signal Specification/1
  Signal Specification/1 -> Terminator/1

== system LunarMicrogrid_Full/BESS Controller/PIctrl/Tsamp - Ngain/External Ts ==
  U : Inport  SampleTime=SampleTime
  Ts : Inport  Port=2  SampleTime=SampleTime
  Ungain*Ts Prod Out : Product  OutMin=UngainTsProdOutMin  OutMax=UngainTsProdOutMax  RndMeth=Simplest  SampleTime=SampleTime
  Out1 : Outport  SampleTime=SampleTime
  wires:
  Ts/1 -> Ungain*Ts Prod Out/2
  Ungain*Ts Prod Out/1 -> Out1/1
  U/1 -> Ungain*Ts Prod Out/1

== system LunarMicrogrid_Full/BESS Controller/PIctrl/Tsamp - Ngain/Passthrough ==
  U : Inport  SampleTime=SampleTime
  Ts : Inport  Port=2  SampleTime=SampleTime
  Terminator : Terminator
  Out1 : Outport  SampleTime=SampleTime
  wires:
  U/1 -> Out1/1
  Ts/1 -> Terminator/1

== system LunarMicrogrid_Full/BESS Controller/PIctrl/postSat Signal/Feedback_Path ==
  feedback : Inport  SampleTime=SampleTime
  forward : Inport  Port=2  SampleTime=SampleTime
  Terminator1 : Terminator
  Out1 : Outport  SampleTime=SampleTime
  wires:
  feedback/1 -> Out1/1
  forward/1 -> Terminator1/1

== system LunarMicrogrid_Full/BESS Controller/PIctrl/postSat Signal/Forward_Path ==
  feedback : Inport  SampleTime=SampleTime
  forward : Inport  Port=2  SampleTime=SampleTime
  Signal Specification1 : SignalSpecification  DisableCoverage=on  OutDataTypeStr=boolean  SampleTime=SampleTime
  Terminator1 : Terminator
  Out1 : Outport  SampleTime=SampleTime
  wires:
  forward/1 -> Out1/1
  feedback/1 -> Signal Specification1/1
  Signal Specification1/1 -> Terminator1/1

== system LunarMicrogrid_Full/BESS Controller/PIctrl/preInt Signal/External PreInt ==
  preInt : Inport  SampleTime=SampleTime
  extAW : Inport  Port=2  SampleTime=SampleTime
  Terminator1 : Terminator
  Out1 : Outport  SampleTime=SampleTime
  wires:
  preInt/1 -> Terminator1/1
  extAW/1 -> Out1/1

== system LunarMicrogrid_Full/BESS Controller/PIctrl/preInt Signal/Internal PreInt ==
  preInt : Inport  SampleTime=SampleTime
  extAW : Inport  Port=2  SampleTime=SampleTime
  Signal Specification1 : SignalSpecification  DisableCoverage=on  OutDataTypeStr=boolean  SampleTime=SampleTime
  Terminator1 : Terminator
  Out1 : Outport  SampleTime=SampleTime
  wires:
  Signal Specification1/1 -> Terminator1/1
  extAW/1 -> Signal Specification1/1
  preInt/1 -> Out1/1

== system LunarMicrogrid_Full/BESS Controller/PIctrl/preSat Signal/Feedback_Path ==
  feedback : Inport  SampleTime=SampleTime
  forward : Inport  Port=2  SampleTime=SampleTime
  Terminator1 : Terminator
  Out1 : Outport  SampleTime=SampleTime
  wires:
  feedback/1 -> Out1/1
  forward/1 -> Terminator1/1

== system LunarMicrogrid_Full/BESS Controller/PIctrl/preSat Signal/Forward_Path ==
  feedback : Inport  SampleTime=SampleTime
  forward : Inport  Port=2  SampleTime=SampleTime
  Signal Specification1 : SignalSpecification  DisableCoverage=on  OutDataTypeStr=boolean  SampleTime=SampleTime
  Terminator1 : Terminator
  Out1 : Outport  SampleTime=SampleTime
  wires:
  forward/1 -> Out1/1
  feedback/1 -> Signal Specification1/1
  Signal Specification1/1 -> Terminator1/1

== system LunarMicrogrid_Full/BESS Controller/DABCtrl2/Anti-windup/Cont. Clamping Ideal/Dead Zone ==
  preSat : Inport
  Upper Limit : Inport  Port=2  SampleTime=SampleTime
  Lower Limit : Inport  Port=3  SampleTime=SampleTime
  Disabled : Subsystem  VariantControl=Disabled
  Enabled : Subsystem  VariantControl=Enabled
  External : Subsystem  VariantControl=External
  DZ out : Outport

== system LunarMicrogrid_Full/BESS Controller/DABCtrl2/Anti-windup/Cont. Clamping Parallel/Dead Zone ==
  preSat : Inport
  Upper Limit : Inport  Port=2  SampleTime=SampleTime
  Lower Limit : Inport  Port=3  SampleTime=SampleTime
  Disabled : Subsystem  VariantControl=Disabled
  Enabled : Subsystem  VariantControl=Enabled
  External : Subsystem  VariantControl=External
  DZ out : Outport

== system LunarMicrogrid_Full/BESS Controller/DABCtrl2/Anti-windup/Disc. Clamping Ideal/Dead Zone ==
  preSat : Inport
  Upper Limit : Inport  Port=2  SampleTime=SampleTime
  Lower Limit : Inport  Port=3  SampleTime=SampleTime
  Disabled : Subsystem  VariantControl=Disabled
  Enabled : Subsystem  VariantControl=Enabled
  External : Subsystem  VariantControl=External
  DZ out : Outport

== system LunarMicrogrid_Full/BESS Controller/DABCtrl2/Anti-windup/Disc. Clamping Parallel/Dead Zone ==
  preSat : Inport
  Upper Limit : Inport  Port=2  SampleTime=SampleTime
  Lower Limit : Inport  Port=3  SampleTime=SampleTime
  Disabled : Subsystem  VariantControl=Disabled
  Enabled : Subsystem  VariantControl=Enabled
  External : Subsystem  VariantControl=External
  DZ out : Outport

== system LunarMicrogrid_Full/BESS Controller/DABCtrl2/Filter/Differentiator/Tsamp ==
  U : Inport  SampleTime=SampleTime
  Ts : Inport  Port=2  SampleTime=SampleTime
  External Ts : Subsystem  VariantControl=ExternalTs
  Internal Ts : Subsystem  VariantControl=InternalTs
  Out1 : Outport  SampleTime=SampleTime

== system LunarMicrogrid_Full/BESS Controller/DABCtrl2/Filter/Disc. Backward Euler Filter/Tsamp ==
  N : Inport  SampleTime=SampleTime
  Ts : Inport  Port=2  SampleTime=SampleTime
  External Ts : Subsystem  VariantControl=ExternalTs
  Internal Ts : Subsystem  VariantControl=InternalTs
  Out1 : Outport  SampleTime=SampleTime

== system LunarMicrogrid_Full/BESS Controller/DABCtrl2/Filter/Disc. Backward Euler Filter Only/Tsamp ==
  N : Inport  SampleTime=SampleTime
  Ts : Inport  Port=2  SampleTime=SampleTime
  External Ts : Subsystem  VariantControl=ExternalTs
  Internal Ts : Subsystem  VariantControl=InternalTs
  Out1 : Outport  SampleTime=SampleTime

== system LunarMicrogrid_Full/BESS Controller/DABCtrl2/Filter/Disc. Trapezoidal Filter/Tsamp ==
  N : Inport  SampleTime=SampleTime
  Ts : Inport  Port=2  SampleTime=SampleTime
  External Ts : Subsystem  VariantControl=ExternalTs
  Internal Ts : Subsystem  VariantControl=InternalTs
  Out1 : Outport  SampleTime=SampleTime

== system LunarMicrogrid_Full/BESS Controller/DABCtrl2/Filter/Disc. Trapezoidal Filter Only/Tsamp ==
  N : Inport  SampleTime=SampleTime
  Ts : Inport  Port=2  SampleTime=SampleTime
  External Ts : Subsystem  VariantControl=ExternalTs
  Internal Ts : Subsystem  VariantControl=InternalTs
  Out1 : Outport  SampleTime=SampleTime

== system LunarMicrogrid_Full/BESS Controller/PIctrl/Anti-windup/Cont. Clamping Ideal/Dead Zone ==
  preSat : Inport
  Upper Limit : Inport  Port=2  SampleTime=SampleTime
  Lower Limit : Inport  Port=3  SampleTime=SampleTime
  Disabled : Subsystem  VariantControl=Disabled
  Enabled : Subsystem  VariantControl=Enabled
  External : Subsystem  VariantControl=External
  DZ out : Outport

== system LunarMicrogrid_Full/BESS Controller/PIctrl/Anti-windup/Cont. Clamping Parallel/Dead Zone ==
  preSat : Inport
  Upper Limit : Inport  Port=2  SampleTime=SampleTime
  Lower Limit : Inport  Port=3  SampleTime=SampleTime
  Disabled : Subsystem  VariantControl=Disabled
  Enabled : Subsystem  VariantControl=Enabled
  External : Subsystem  VariantControl=External
  DZ out : Outport

== system LunarMicrogrid_Full/BESS Controller/PIctrl/Anti-windup/Disc. Clamping Ideal/Dead Zone ==
  preSat : Inport
  Upper Limit : Inport  Port=2  SampleTime=SampleTime
  Lower Limit : Inport  Port=3  SampleTime=SampleTime
  Disabled : Subsystem  VariantControl=Disabled
  Enabled : Subsystem  VariantControl=Enabled
  External : Subsystem  VariantControl=External
  DZ out : Outport

== system LunarMicrogrid_Full/BESS Controller/PIctrl/Anti-windup/Disc. Clamping Parallel/Dead Zone ==
  preSat : Inport
  Upper Limit : Inport  Port=2  SampleTime=SampleTime
  Lower Limit : Inport  Port=3  SampleTime=SampleTime
  Disabled : Subsystem  VariantControl=Disabled
  Enabled : Subsystem  VariantControl=Enabled
  External : Subsystem  VariantControl=External
  DZ out : Outport

== system LunarMicrogrid_Full/BESS Controller/PIctrl/Filter/Differentiator/Tsamp ==
  U : Inport  SampleTime=SampleTime
  Ts : Inport  Port=2  SampleTime=SampleTime
  External Ts : Subsystem  VariantControl=ExternalTs
  Internal Ts : Subsystem  VariantControl=InternalTs
  Out1 : Outport  SampleTime=SampleTime

== system LunarMicrogrid_Full/BESS Controller/PIctrl/Filter/Disc. Backward Euler Filter/Tsamp ==
  N : Inport  SampleTime=SampleTime
  Ts : Inport  Port=2  SampleTime=SampleTime
  External Ts : Subsystem  VariantControl=ExternalTs
  Internal Ts : Subsystem  VariantControl=InternalTs
  Out1 : Outport  SampleTime=SampleTime

== system LunarMicrogrid_Full/BESS Controller/PIctrl/Filter/Disc. Backward Euler Filter Only/Tsamp ==
  N : Inport  SampleTime=SampleTime
  Ts : Inport  Port=2  SampleTime=SampleTime
  External Ts : Subsystem  VariantControl=ExternalTs
  Internal Ts : Subsystem  VariantControl=InternalTs
  Out1 : Outport  SampleTime=SampleTime

== system LunarMicrogrid_Full/BESS Controller/PIctrl/Filter/Disc. Trapezoidal Filter/Tsamp ==
  N : Inport  SampleTime=SampleTime
  Ts : Inport  Port=2  SampleTime=SampleTime
  External Ts : Subsystem  VariantControl=ExternalTs
  Internal Ts : Subsystem  VariantControl=InternalTs
  Out1 : Outport  SampleTime=SampleTime

== system LunarMicrogrid_Full/BESS Controller/PIctrl/Filter/Disc. Trapezoidal Filter Only/Tsamp ==
  N : Inport  SampleTime=SampleTime
  Ts : Inport  Port=2  SampleTime=SampleTime
  External Ts : Subsystem  VariantControl=ExternalTs
  Internal Ts : Subsystem  VariantControl=InternalTs
  Out1 : Outport  SampleTime=SampleTime

== system LunarMicrogrid_Full/BESS Controller/DABCtrl2/Anti-windup/Cont. Clamping Ideal/Dead Zone/Disabled ==

== system LunarMicrogrid_Full/BESS Controller/DABCtrl2/Anti-windup/Cont. Clamping Ideal/Dead Zone/Enabled ==
  preSat : Inport
  DeadZone : DeadZone  DisableCoverage=on  LowerValue=LowerSaturationLimit  UpperValue=UpperSaturationLimit  LinearizeAsGain=off  SaturateOnIntegerOverflow=off
  DZ out : Outport
  wires:
  preSat/1 -> DeadZone/1
  DeadZone/1 -> DZ out/1

== system LunarMicrogrid_Full/BESS Controller/DABCtrl2/Anti-windup/Cont. Clamping Ideal/Dead Zone/External ==
  preSat : Inport
  Upper Limit : Inport  Port=2  SampleTime=SampleTime
  Lower Limit : Inport  Port=3  SampleTime=SampleTime
  Dead Zone Dynamic1 : sl_discontinuities/Dead Zone Dynamic
  DZ out : Outport
  wires:
  preSat/1 -> Dead Zone Dynamic1/2
  Lower Limit/1 -> Dead Zone Dynamic1/3
  Upper Limit/1 -> Dead Zone Dynamic1/1
  Dead Zone Dynamic1/1 -> DZ out/1

== system LunarMicrogrid_Full/BESS Controller/DABCtrl2/Anti-windup/Cont. Clamping Parallel/Dead Zone/Disabled ==

== system LunarMicrogrid_Full/BESS Controller/DABCtrl2/Anti-windup/Cont. Clamping Parallel/Dead Zone/Enabled ==
  preSat : Inport
  DeadZone : DeadZone  DisableCoverage=on  LowerValue=LowerSaturationLimit  UpperValue=UpperSaturationLimit  LinearizeAsGain=off  SaturateOnIntegerOverflow=off
  DZ out : Outport
  wires:
  preSat/1 -> DeadZone/1
  DeadZone/1 -> DZ out/1

== system LunarMicrogrid_Full/BESS Controller/DABCtrl2/Anti-windup/Cont. Clamping Parallel/Dead Zone/External ==
  preSat : Inport
  Upper Limit : Inport  Port=2  SampleTime=SampleTime
  Lower Limit : Inport  Port=3  SampleTime=SampleTime
  Dead Zone Dynamic : sl_discontinuities/Dead Zone Dynamic
  DZ out : Outport
  wires:
  preSat/1 -> Dead Zone Dynamic/2
  Lower Limit/1 -> Dead Zone Dynamic/3
  Upper Limit/1 -> Dead Zone Dynamic/1
  Dead Zone Dynamic/1 -> DZ out/1

== system LunarMicrogrid_Full/BESS Controller/DABCtrl2/Anti-windup/Disc. Clamping Ideal/Dead Zone/Disabled ==

== system LunarMicrogrid_Full/BESS Controller/DABCtrl2/Anti-windup/Disc. Clamping Ideal/Dead Zone/Enabled ==
  preSat : Inport
  DeadZone : DeadZone  DisableCoverage=on  LowerValue=LowerSaturationLimit  UpperValue=UpperSaturationLimit  LinearizeAsGain=off  SaturateOnIntegerOverflow=off
  DZ out : Outport
  wires:
  DeadZone/1 -> DZ out/1
  preSat/1 -> DeadZone/1

== system LunarMicrogrid_Full/BESS Controller/DABCtrl2/Anti-windup/Disc. Clamping Ideal/Dead Zone/External ==
  preSat : Inport
  Upper Limit : Inport  Port=2  SampleTime=SampleTime
  Lower Limit : Inport  Port=3  SampleTime=SampleTime
  Dead Zone Dynamic : sl_discontinuities/Dead Zone Dynamic
  DZ out : Outport
  wires:
  Dead Zone Dynamic/1 -> DZ out/1
  Upper Limit/1 -> Dead Zone Dynamic/1
  Lower Limit/1 -> Dead Zone Dynamic/3
  preSat/1 -> Dead Zone Dynamic/2

== system LunarMicrogrid_Full/BESS Controller/DABCtrl2/Anti-windup/Disc. Clamping Parallel/Dead Zone/Disabled ==

== system LunarMicrogrid_Full/BESS Controller/DABCtrl2/Anti-windup/Disc. Clamping Parallel/Dead Zone/Enabled ==
  preSat : Inport
  DeadZone : DeadZone  DisableCoverage=on  LowerValue=LowerSaturationLimit  UpperValue=UpperSaturationLimit  LinearizeAsGain=off  SaturateOnIntegerOverflow=off
  DZ out : Outport
  wires:
  DeadZone/1 -> DZ out/1
  preSat/1 -> DeadZone/1

== system LunarMicrogrid_Full/BESS Controller/DABCtrl2/Anti-windup/Disc. Clamping Parallel/Dead Zone/External ==
  preSat : Inport
  Upper Limit : Inport  Port=2  SampleTime=SampleTime
  Lower Limit : Inport  Port=3  SampleTime=SampleTime
  Dead Zone Dynamic : sl_discontinuities/Dead Zone Dynamic
  DZ out : Outport
  wires:
  Dead Zone Dynamic/1 -> DZ out/1
  Upper Limit/1 -> Dead Zone Dynamic/1
  Lower Limit/1 -> Dead Zone Dynamic/3
  preSat/1 -> Dead Zone Dynamic/2
